simulink model "Assembly_For_Simscape"  (R2023b)
settings: Solver=VariableStepAuto  StartTime=0.0  StopTime=38  RelTol=1e-3
InitFcn:
  | addpath(genpath(pwd));
  | disp('✅ InitFcn executed');
  | Assembly_For_Simscape_DataFile;  % Run the data file script to load smiData
model workspace: external: MAT-File C:\Users\amine\OneDrive - TUM\Desktop\Bachelor Thesis\SIMSCAPE\Simscape files\slprj\sim\varcache\Assembly_For_Simscape\varInfo.mat (data not in the file)
undefined symbols (not defined in the file or in its folder): sigbuilder_block, smiData, X, Y, Z
libraries: sm_lib x76, nesl_utility x32
(part 3 of 3)

== system Assembly_For_Simscape/Project_MiniHex/Stewart_Platform/Horn-BallJoint-Rod-BallJoint 4/ASSEMBLY_Horn_sphere_1_RIGID ==
  ReferenceFrame : sm_lib/Frames and Transforms/Reference Frame
  Solid : sm_lib/Body Elements/File Solid  ExtGeomFileName=ASSEMBLY_Horn_sphere_Default_sldprt.STEP  UnitType=FromFile  ExtGeomFileUnits=m  StepReaderType=HEX  ExportConvexHullGeometry=off  InertiaType=Custom  Mass=smiData.Solid(4).mass  MassUnits=kg  CenterOfMass=smiData.Solid(4).CoM  CenterOfMassUnits=mm  MomentsOfInertia=smiData.Solid(4).MoI  MomentsOfInertiaUnits=kg*mm^2  ProductsOfInertia=smiData.Solid(4).PoI  ProductsOfInertiaUnits=kg*mm^2  BasedOnType=DensityFromFile  Density=1000  DensityUnits=kg/m^3  DoExposeReferenceFrame=off  SerializedFrames=<Frames><Frame><Id>Frame1</Id><Value><Name>horn central frame 2</Name><Origin><Source>GeometricFeature</Source><FeatureName>circular curve 6</FeatureName></Origin><PrimaryAxis><DefinedDirection>+Z</DefinedDirection><Source>CenterOfMassFrame</Source><SourceDirection>-Z</SourceDirection><FeatureName></FeatureName></PrimaryAxis><SecondaryAxis><DefinedDirection>-X</DefinedDirection><Source>CenterOfMassFrame</Source><SourceDirection>+X</SourceDirection><FeatureName></FeatureName></SecondaryAxis></Value></Frame><Frame><Id>Frame2</Id><Value><Name>horn outer frame 2</Name><Origin><Source>GeometricFeature</Source><FeatureName>circular curve 79</FeatureName></Origin><PrimaryAxis><DefinedDirection>+Z</DefinedDirection><Source>CenterOfMassFrame</Source><SourceDirection>-Z</SourceDirection><FeatureName></FeatureName></PrimaryAxis><SecondaryAxis><DefinedDirection>+X</DefinedDirection><Source>GeometricFeature</Source><SourceDirection>+X</SourceDirection><FeatureName>circular curve 79</FeatureName></SecondaryAxis></Value></Frame><Frame><Id>Frame3</Id><Value><Name>COG</Name><Origin><Source>CenterOfMassFrame</Source><FeatureName></FeatureName></Origin><PrimaryAxis><DefinedDirection>-Z</DefinedDirection><Source>GeometricFeature</Source><SourceDirection>+Z</SourceDirection><FeatureName>planar surface 3</FeatureName></PrimaryAxis><SecondaryAxis><DefinedDirection>+X</DefinedDirection><Source>CenterOfMassFrame</Source><SourceDirection>+X</SourceDirection><FeatureName></FeatureName></SecondaryAxis></Value></Frame></Frames>  GraphicType=FromGeometry  MarkerShape=Sphere  MarkerSize=10  GraphicVisPropType=SimpleVisualProperties  GraphicDiffuseColor=smiData.Solid(4).color  GraphicSpecularColor=[0.5 0.5 0.5 1.0]  GraphicAmbientColor=[0.15 0.15 0.15 1.0]  GraphicEmissiveColor=[0.0 0.0 0.0 1.0]  GraphicShininess=75  GraphicOpacity=smiData.Solid(4).opacity
  F2 : PMIOPort  Side=Left
  F1 : PMIOPort  Port=2  Side=Left
  F : PMIOPort  Port=3  Side=Left
  connections:
  ReferenceFrame/RConn1 -- F2/RConn1 -- Solid/LConn2
  Solid/LConn1 -- F1/RConn1
  Solid/RConn1 -- F/RConn1

== system Assembly_For_Simscape/Project_MiniHex/Stewart_Platform/Horn-BallJoint-Rod-BallJoint 4/Ball_Joint_3mm_outer_sphere_2_RIGID ==
  ReferenceFrame : sm_lib/Frames and Transforms/Reference Frame
  Solid : sm_lib/Body Elements/File Solid  ExtGeomFileName=Ball Joint 3mm outer sphere_Default_sldprt.STEP  UnitType=FromFile  ExtGeomFileUnits=m  StepReaderType=HEX  ExportConvexHullGeometry=off  InertiaType=Custom  Mass=smiData.Solid(5).mass  MassUnits=kg  CenterOfMass=smiData.Solid(5).CoM  CenterOfMassUnits=mm  MomentsOfInertia=smiData.Solid(5).MoI  MomentsOfInertiaUnits=kg*mm^2  ProductsOfInertia=smiData.Solid(5).PoI  ProductsOfInertiaUnits=kg*mm^2  BasedOnType=DensityFromFile  Density=1000  DensityUnits=kg/m^3  DoExposeReferenceFrame=on  SerializedFrames=<Frames><Frame><Id>Frame1</Id><Value><Name>ball joint center</Name><Origin><Source>GeometricFeature</Source><FeatureName>spherical surface 4</FeatureName></Origin><PrimaryAxis><DefinedDirection>+Z</DefinedDirection><Source>GeometricFeature</Source><SourceDirection>+Z</SourceDirection><FeatureName>circular curve 27</FeatureName></PrimaryAxis><SecondaryAxis><DefinedDirection>-Y</DefinedDirection><Source>ReferenceFrame</Source><SourceDirection>+Y</SourceDirection><FeatureName></FeatureName></SecondaryAxis></Value></Frame><Frame><Id>Frame2</Id><Value><Name>Rod rotation link</Name><Origin><Source>GeometricFeature</Source><FeatureName>planar surface 3</FeatureName></Origin><PrimaryAxis><DefinedDirection>+Z</DefinedDirection><Source>GeometricFeature</Source><SourceDirection>+Z</SourceDirection><FeatureName>planar surface 3</FeatureName></PrimaryAxis><SecondaryAxis><DefinedDirection>+X</DefinedDirection><Source>ReferenceFrame</Source><SourceDirection>+X</SourceDirection><FeatureName></FeatureName></SecondaryAxis></Value></Frame></Frames>  GraphicType=FromGeometry  MarkerShape=Sphere  MarkerSize=10  GraphicVisPropType=SimpleVisualProperties  GraphicDiffuseColor=smiData.Solid(5).color  GraphicSpecularColor=[0.5 0.5 0.5 1.0]  GraphicAmbientColor=[0.15 0.15 0.15 1.0]  GraphicEmissiveColor=[0.0 0.0 0.0 1.0]  GraphicShininess=75  GraphicOpacity=smiData.Solid(5).opacity
  F : PMIOPort  Side=Left
  F1 : PMIOPort  Port=2  Side=Left
  connections:
  ReferenceFrame/RConn1 -- Solid/RConn1
  Solid/LConn1 -- F/RConn1
  Solid/LConn2 -- F1/RConn1

== system Assembly_For_Simscape/Project_MiniHex/Stewart_Platform/Horn-BallJoint-Rod-BallJoint 4/Ball_Joint_3mm_outer_sphere_2_RIGID2 ==
  ReferenceFrame : sm_lib/Frames and Transforms/Reference Frame
  Solid : sm_lib/Body Elements/File Solid  ExtGeomFileName=Ball Joint 3mm outer sphere_Default_sldprt.STEP  UnitType=FromFile  ExtGeomFileUnits=m  StepReaderType=HEX  ExportConvexHullGeometry=off  InertiaType=Custom  Mass=smiData.Solid(5).mass  MassUnits=kg  CenterOfMass=smiData.Solid(5).CoM  CenterOfMassUnits=mm  MomentsOfInertia=smiData.Solid(5).MoI  MomentsOfInertiaUnits=kg*mm^2  ProductsOfInertia=smiData.Solid(5).PoI  ProductsOfInertiaUnits=kg*mm^2  BasedOnType=DensityFromFile  Density=1000  DensityUnits=kg/m^3  DoExposeReferenceFrame=on  SerializedFrames=<Frames><Frame><Id>Frame1</Id><Value><Name>ball joint center</Name><Origin><Source>GeometricFeature</Source><FeatureName>spherical surface 4</FeatureName></Origin><PrimaryAxis><DefinedDirection>+Z</DefinedDirection><Source>GeometricFeature</Source><SourceDirection>+Z</SourceDirection><FeatureName>circular curve 27</FeatureName></PrimaryAxis><SecondaryAxis><DefinedDirection>-Y</DefinedDirection><Source>ReferenceFrame</Source><SourceDirection>+Y</SourceDirection><FeatureName></FeatureName></SecondaryAxis></Value></Frame><Frame><Id>Frame2</Id><Value><Name>Rod rotation link</Name><Origin><Source>GeometricFeature</Source><FeatureName>planar surface 3</FeatureName></Origin><PrimaryAxis><DefinedDirection>+Z</DefinedDirection><Source>GeometricFeature</Source><SourceDirection>+Z</SourceDirection><FeatureName>planar surface 3</FeatureName></PrimaryAxis><SecondaryAxis><DefinedDirection>+X</DefinedDirection><Source>ReferenceFrame</Source><SourceDirection>+X</SourceDirection><FeatureName></FeatureName></SecondaryAxis></Value></Frame></Frames>  GraphicType=FromGeometry  MarkerShape=Sphere  MarkerSize=10  GraphicVisPropType=SimpleVisualProperties  GraphicDiffuseColor=smiData.Solid(5).color  GraphicSpecularColor=[0.5 0.5 0.5 1.0]  GraphicAmbientColor=[0.15 0.15 0.15 1.0]  GraphicEmissiveColor=[0.0 0.0 0.0 1.0]  GraphicShininess=75  GraphicOpacity=smiData.Solid(5).opacity
  F : PMIOPort  Side=Left
  F1 : PMIOPort  Port=2  Side=Right
  connections:
  ReferenceFrame/RConn1 -- Solid/RConn1
  Solid/LConn1 -- F/RConn1
  Solid/LConn2 -- F1/RConn1

== system Assembly_For_Simscape/Project_MiniHex/Stewart_Platform/Horn-BallJoint-Rod-BallJoint 4/Rod_1_RIGID ==
  ReferenceFrame : sm_lib/Frames and Transforms/Reference Frame
  Solid : sm_lib/Body Elements/File Solid  ExtGeomFileName=Rod_Default_sldprt.STEP  UnitType=FromFile  ExtGeomFileUnits=m  StepReaderType=HEX  ExportConvexHullGeometry=off  InertiaType=Custom  Mass=smiData.Solid(3).mass  MassUnits=kg  CenterOfMass=smiData.Solid(3).CoM  CenterOfMassUnits=m  MomentsOfInertia=smiData.Solid(3).MoI  MomentsOfInertiaUnits=kg*m^2  ProductsOfInertia=smiData.Solid(3).PoI  ProductsOfInertiaUnits=kg*m^2  BasedOnType=DensityFromFile  Density=1000  DensityUnits=kg/m^3  DoExposeReferenceFrame=on  SerializedFrames=<Frames><Frame><Id>Frame1</Id><Value><Name>F1</Name><Origin><Source>GeometricFeature</Source><FeatureName>planar surface 4</FeatureName></Origin><PrimaryAxis><DefinedDirection>-Z</DefinedDirection><Source>GeometricFeature</Source><SourceDirection>+Z</SourceDirection><FeatureName>planar surface 4</FeatureName></PrimaryAxis><SecondaryAxis><DefinedDirection>+X</DefinedDirection><Source>ReferenceFrame</Source><SourceDirection>+X</SourceDirection><FeatureName></FeatureName></SecondaryAxis></Value></Frame><Frame><Id>Frame2</Id><Value><Name>F2</Name><Origin><Source>GeometricFeature</Source><FeatureName>planar surface 3</FeatureName></Origin><PrimaryAxis><DefinedDirection>-Z</DefinedDirection><Source>CenterOfMassFrame</Source><SourceDirection>+Y</SourceDirection><FeatureName></FeatureName></PrimaryAxis><SecondaryAxis><DefinedDirection>+Y</DefinedDirection><Source>CenterOfMassFrame</Source><SourceDirection>+Z</SourceDirection><FeatureName></FeatureName></SecondaryAxis></Value></Frame></Frames>  GraphicType=FromGeometry  MarkerShape=Sphere  MarkerSize=10  GraphicVisPropType=SimpleVisualProperties  GraphicDiffuseColor=smiData.Solid(3).color  GraphicSpecularColor=[0.5 0.5 0.5 1.0]  GraphicAmbientColor=[0.15 0.15 0.15 1.0]  GraphicEmissiveColor=[0.0 0.0 0.0 1.0]  GraphicShininess=75  GraphicOpacity=smiData.Solid(3).opacity
  F : PMIOPort  Side=Left
  F1 : PMIOPort  Port=2  Side=Right
  connections:
  ReferenceFrame/RConn1 -- Solid/RConn1
  Solid/LConn1 -- F/RConn1
  Solid/LConn2 -- F1/RConn1

== system Assembly_For_Simscape/Project_MiniHex/Stewart_Platform/Horn-BallJoint-Rod-BallJoint 5/ASSEMBLY_Horn_sphere_1_RIGID ==
  ReferenceFrame : sm_lib/Frames and Transforms/Reference Frame
  Solid : sm_lib/Body Elements/File Solid  ExtGeomFileName=ASSEMBLY_Horn_sphere_Default_sldprt.STEP  UnitType=FromFile  ExtGeomFileUnits=m  StepReaderType=HEX  ExportConvexHullGeometry=off  InertiaType=Custom  Mass=smiData.Solid(4).mass  MassUnits=kg  CenterOfMass=smiData.Solid(4).CoM  CenterOfMassUnits=mm  MomentsOfInertia=smiData.Solid(4).MoI  MomentsOfInertiaUnits=kg*mm^2  ProductsOfInertia=smiData.Solid(4).PoI  ProductsOfInertiaUnits=kg*mm^2  BasedOnType=DensityFromFile  Density=1000  DensityUnits=kg/m^3  DoExposeReferenceFrame=off  SerializedFrames=<Frames><Frame><Id>Frame1</Id><Value><Name>horn central frame</Name><Origin><Source>GeometricFeature</Source><FeatureName>circular curve 6</FeatureName></Origin><PrimaryAxis><DefinedDirection>+Z</DefinedDirection><Source>CenterOfMassFrame</Source><SourceDirection>-Z</SourceDirection><FeatureName></FeatureName></PrimaryAxis><SecondaryAxis><DefinedDirection>-X</DefinedDirection><Source>CenterOfMassFrame</Source><SourceDirection>-X</SourceDirection><FeatureName></FeatureName></SecondaryAxis></Value></Frame><Frame><Id>Frame2</Id><Value><Name>horn outer frame </Name><Origin><Source>GeometricFeature</Source><FeatureName>circular curve 79</FeatureName></Origin><PrimaryAxis><DefinedDirection>+Z</DefinedDirection><Source>CenterOfMassFrame</Source><SourceDirection>-Z</SourceDirection><FeatureName></FeatureName></PrimaryAxis><SecondaryAxis><DefinedDirection>-X</DefinedDirection><Source>GeometricFeature</Source><SourceDirection>+X</SourceDirection><FeatureName>circular curve 79</FeatureName></SecondaryAxis></Value></Frame><Frame><Id>Frame3</Id><Value><Name>COG</Name><Origin><Source>CenterOfMassFrame</Source><FeatureName></FeatureName></Origin><PrimaryAxis><DefinedDirection>-Z</DefinedDirection><Source>GeometricFeature</Source><SourceDirection>+Z</SourceDirection><FeatureName>planar surface 3</FeatureName></PrimaryAxis><SecondaryAxis><DefinedDirection>+X</DefinedDirection><Source>CenterOfMassFrame</Source><SourceDirection>+X</SourceDirection><FeatureName></FeatureName></SecondaryAxis></Value></Frame></Frames>  GraphicType=FromGeometry  MarkerShape=Sphere  MarkerSize=10  GraphicVisPropType=SimpleVisualProperties  GraphicDiffuseColor=smiData.Solid(4).color  GraphicSpecularColor=[0.5 0.5 0.5 1.0]  GraphicAmbientColor=[0.15 0.15 0.15 1.0]  GraphicEmissiveColor=[0.0 0.0 0.0 1.0]  GraphicShininess=75  GraphicOpacity=smiData.Solid(4).opacity
  F2 : PMIOPort  Side=Left
  F1 : PMIOPort  Port=2  Side=Left
  F : PMIOPort  Port=3  Side=Left
  connections:
  ReferenceFrame/RConn1 -- Solid/LConn2 -- F2/RConn1
  Solid/LConn1 -- F1/RConn1
  Solid/RConn1 -- F/RConn1

== system Assembly_For_Simscape/Project_MiniHex/Stewart_Platform/Horn-BallJoint-Rod-BallJoint 5/Ball_Joint_3mm_outer_sphere_2_RIGID ==
  ReferenceFrame : sm_lib/Frames and Transforms/Reference Frame
  Solid : sm_lib/Body Elements/File Solid  ExtGeomFileName=Ball Joint 3mm outer sphere_Default_sldprt.STEP  UnitType=FromFile  ExtGeomFileUnits=m  StepReaderType=HEX  ExportConvexHullGeometry=off  InertiaType=Custom  Mass=smiData.Solid(5).mass  MassUnits=kg  CenterOfMass=smiData.Solid(5).CoM  CenterOfMassUnits=mm  MomentsOfInertia=smiData.Solid(5).MoI  MomentsOfInertiaUnits=kg*mm^2  ProductsOfInertia=smiData.Solid(5).PoI  ProductsOfInertiaUnits=kg*mm^2  BasedOnType=DensityFromFile  Density=1000  DensityUnits=kg/m^3  DoExposeReferenceFrame=on  SerializedFrames=<Frames><Frame><Id>Frame1</Id><Value><Name>ball joint center</Name><Origin><Source>GeometricFeature</Source><FeatureName>spherical surface 4</FeatureName></Origin><PrimaryAxis><DefinedDirection>+Z</DefinedDirection><Source>GeometricFeature</Source><SourceDirection>+Z</SourceDirection><FeatureName>circular curve 27</FeatureName></PrimaryAxis><SecondaryAxis><DefinedDirection>-Y</DefinedDirection><Source>ReferenceFrame</Source><SourceDirection>+Y</SourceDirection><FeatureName></FeatureName></SecondaryAxis></Value></Frame><Frame><Id>Frame2</Id><Value><Name>Rod rotation link</Name><Origin><Source>GeometricFeature</Source><FeatureName>planar surface 3</FeatureName></Origin><PrimaryAxis><DefinedDirection>+Z</DefinedDirection><Source>GeometricFeature</Source><SourceDirection>+Z</SourceDirection><FeatureName>planar surface 3</FeatureName></PrimaryAxis><SecondaryAxis><DefinedDirection>+X</DefinedDirection><Source>ReferenceFrame</Source><SourceDirection>+X</SourceDirection><FeatureName></FeatureName></SecondaryAxis></Value></Frame></Frames>  GraphicType=FromGeometry  MarkerShape=Sphere  MarkerSize=10  GraphicVisPropType=SimpleVisualProperties  GraphicDiffuseColor=smiData.Solid(5).color  GraphicSpecularColor=[0.5 0.5 0.5 1.0]  GraphicAmbientColor=[0.15 0.15 0.15 1.0]  GraphicEmissiveColor=[0.0 0.0 0.0 1.0]  GraphicShininess=75  GraphicOpacity=smiData.Solid(5).opacity
  F : PMIOPort  Side=Left
  F1 : PMIOPort  Port=2  Side=Left
  connections:
  ReferenceFrame/RConn1 -- Solid/RConn1
  Solid/LConn1 -- F/RConn1
  Solid/LConn2 -- F1/RConn1

== system Assembly_For_Simscape/Project_MiniHex/Stewart_Platform/Horn-BallJoint-Rod-BallJoint 5/Ball_Joint_3mm_outer_sphere_2_RIGID2 ==
  ReferenceFrame : sm_lib/Frames and Transforms/Reference Frame
  Solid : sm_lib/Body Elements/File Solid  ExtGeomFileName=Ball Joint 3mm outer sphere_Default_sldprt.STEP  UnitType=FromFile  ExtGeomFileUnits=m  StepReaderType=HEX  ExportConvexHullGeometry=off  InertiaType=Custom  Mass=smiData.Solid(5).mass  MassUnits=kg  CenterOfMass=smiData.Solid(5).CoM  CenterOfMassUnits=mm  MomentsOfInertia=smiData.Solid(5).MoI  MomentsOfInertiaUnits=kg*mm^2  ProductsOfInertia=smiData.Solid(5).PoI  ProductsOfInertiaUnits=kg*mm^2  BasedOnType=DensityFromFile  Density=1000  DensityUnits=kg/m^3  DoExposeReferenceFrame=on  SerializedFrames=<Frames><Frame><Id>Frame1</Id><Value><Name>ball joint center</Name><Origin><Source>GeometricFeature</Source><FeatureName>spherical surface 4</FeatureName></Origin><PrimaryAxis><DefinedDirection>+Z</DefinedDirection><Source>GeometricFeature</Source><SourceDirection>+Z</SourceDirection><FeatureName>circular curve 27</FeatureName></PrimaryAxis><SecondaryAxis><DefinedDirection>-Y</DefinedDirection><Source>ReferenceFrame</Source><SourceDirection>+Y</SourceDirection><FeatureName></FeatureName></SecondaryAxis></Value></Frame><Frame><Id>Frame2</Id><Value><Name>Rod rotation link</Name><Origin><Source>GeometricFeature</Source><FeatureName>planar surface 3</FeatureName></Origin><PrimaryAxis><DefinedDirection>+Z</DefinedDirection><Source>GeometricFeature</Source><SourceDirection>+Z</SourceDirection><FeatureName>planar surface 3</FeatureName></PrimaryAxis><SecondaryAxis><DefinedDirection>+X</DefinedDirection><Source>ReferenceFrame</Source><SourceDirection>+X</SourceDirection><FeatureName></FeatureName></SecondaryAxis></Value></Frame></Frames>  GraphicType=FromGeometry  MarkerShape=Sphere  MarkerSize=10  GraphicVisPropType=SimpleVisualProperties  GraphicDiffuseColor=smiData.Solid(5).color  GraphicSpecularColor=[0.5 0.5 0.5 1.0]  GraphicAmbientColor=[0.15 0.15 0.15 1.0]  GraphicEmissiveColor=[0.0 0.0 0.0 1.0]  GraphicShininess=75  GraphicOpacity=smiData.Solid(5).opacity
  F : PMIOPort  Side=Left
  F1 : PMIOPort  Port=2  Side=Right
  connections:
  ReferenceFrame/RConn1 -- Solid/RConn1
  Solid/LConn1 -- F/RConn1
  Solid/LConn2 -- F1/RConn1

== system Assembly_For_Simscape/Project_MiniHex/Stewart_Platform/Horn-BallJoint-Rod-BallJoint 5/Rod_1_RIGID ==
  ReferenceFrame : sm_lib/Frames and Transforms/Reference Frame
  Solid : sm_lib/Body Elements/File Solid  ExtGeomFileName=Rod_Default_sldprt.STEP  UnitType=FromFile  ExtGeomFileUnits=m  StepReaderType=HEX  ExportConvexHullGeometry=off  InertiaType=Custom  Mass=smiData.Solid(3).mass  MassUnits=kg  CenterOfMass=smiData.Solid(3).CoM  CenterOfMassUnits=m  MomentsOfInertia=smiData.Solid(3).MoI  MomentsOfInertiaUnits=kg*m^2  ProductsOfInertia=smiData.Solid(3).PoI  ProductsOfInertiaUnits=kg*m^2  BasedOnType=DensityFromFile  Density=1000  DensityUnits=kg/m^3  DoExposeReferenceFrame=on  SerializedFrames=<Frames><Frame><Id>Frame1</Id><Value><Name>F1</Name><Origin><Source>GeometricFeature</Source><FeatureName>planar surface 4</FeatureName></Origin><PrimaryAxis><DefinedDirection>-Z</DefinedDirection><Source>GeometricFeature</Source><SourceDirection>+Z</SourceDirection><FeatureName>planar surface 4</FeatureName></PrimaryAxis><SecondaryAxis><DefinedDirection>+X</DefinedDirection><Source>ReferenceFrame</Source><SourceDirection>+X</SourceDirection><FeatureName></FeatureName></SecondaryAxis></Value></Frame><Frame><Id>Frame2</Id><Value><Name>F2</Name><Origin><Source>GeometricFeature</Source><FeatureName>planar surface 3</FeatureName></Origin><PrimaryAxis><DefinedDirection>-Z</DefinedDirection><Source>CenterOfMassFrame</Source><SourceDirection>+Y</SourceDirection><FeatureName></FeatureName></PrimaryAxis><SecondaryAxis><DefinedDirection>+Y</DefinedDirection><Source>CenterOfMassFrame</Source><SourceDirection>+Z</SourceDirection><FeatureName></FeatureName></SecondaryAxis></Value></Frame></Frames>  GraphicType=FromGeometry  MarkerShape=Sphere  MarkerSize=10  GraphicVisPropType=SimpleVisualProperties  GraphicDiffuseColor=smiData.Solid(3).color  GraphicSpecularColor=[0.5 0.5 0.5 1.0]  GraphicAmbientColor=[0.15 0.15 0.15 1.0]  GraphicEmissiveColor=[0.0 0.0 0.0 1.0]  GraphicShininess=75  GraphicOpacity=smiData.Solid(3).opacity
  F : PMIOPort  Side=Left
  F1 : PMIOPort  Port=2  Side=Right
  connections:
  ReferenceFrame/RConn1 -- Solid/RConn1
  Solid/LConn1 -- F/RConn1
  Solid/LConn2 -- F1/RConn1

== system Assembly_For_Simscape/Project_MiniHex/Stewart_Platform/Horn-BallJoint-Rod-BallJoint 6/ASSEMBLY_Horn_sphere_1_RIGID ==
  ReferenceFrame : sm_lib/Frames and Transforms/Reference Frame
  Solid : sm_lib/Body Elements/File Solid  ExtGeomFileName=ASSEMBLY_Horn_sphere_Default_sldprt.STEP  UnitType=FromFile  ExtGeomFileUnits=m  StepReaderType=HEX  ExportConvexHullGeometry=off  InertiaType=Custom  Mass=smiData.Solid(4).mass  MassUnits=kg  CenterOfMass=smiData.Solid(4).CoM  CenterOfMassUnits=mm  MomentsOfInertia=smiData.Solid(4).MoI  MomentsOfInertiaUnits=kg*mm^2  ProductsOfInertia=smiData.Solid(4).PoI  ProductsOfInertiaUnits=kg*mm^2  BasedOnType=DensityFromFile  Density=1000  DensityUnits=kg/m^3  DoExposeReferenceFrame=off  SerializedFrames=<Frames><Frame><Id>Frame1</Id><Value><Name>horn central frame 2</Name><Origin><Source>GeometricFeature</Source><FeatureName>circular curve 6</FeatureName></Origin><PrimaryAxis><DefinedDirection>+Z</DefinedDirection><Source>CenterOfMassFrame</Source><SourceDirection>-Z</SourceDirection><FeatureName></FeatureName></PrimaryAxis><SecondaryAxis><DefinedDirection>-X</DefinedDirection><Source>CenterOfMassFrame</Source><SourceDirection>+X</SourceDirection><FeatureName></FeatureName></SecondaryAxis></Value></Frame><Frame><Id>Frame2</Id><Value><Name>horn outer frame 2</Name><Origin><Source>GeometricFeature</Source><FeatureName>circular curve 79</FeatureName></Origin><PrimaryAxis><DefinedDirection>+Z</DefinedDirection><Source>CenterOfMassFrame</Source><SourceDirection>-Z</SourceDirection><FeatureName></FeatureName></PrimaryAxis><SecondaryAxis><DefinedDirection>+X</DefinedDirection><Source>GeometricFeature</Source><SourceDirection>+X</SourceDirection><FeatureName>circular curve 79</FeatureName></SecondaryAxis></Value></Frame><Frame><Id>Frame3</Id><Value><Name>COG</Name><Origin><Source>CenterOfMassFrame</Source><FeatureName></FeatureName></Origin><PrimaryAxis><DefinedDirection>-Z</DefinedDirection><Source>GeometricFeature</Source><SourceDirection>+Z</SourceDirection><FeatureName>planar surface 3</FeatureName></PrimaryAxis><SecondaryAxis><DefinedDirection>+X</DefinedDirection><Source>CenterOfMassFrame</Source><SourceDirection>+X</SourceDirection><FeatureName></FeatureName></SecondaryAxis></Value></Frame></Frames>  GraphicType=FromGeometry  MarkerShape=Sphere  MarkerSize=10  GraphicVisPropType=SimpleVisualProperties  GraphicDiffuseColor=smiData.Solid(4).color  GraphicSpecularColor=[0.5 0.5 0.5 1.0]  GraphicAmbientColor=[0.15 0.15 0.15 1.0]  GraphicEmissiveColor=[0.0 0.0 0.0 1.0]  GraphicShininess=75  GraphicOpacity=smiData.Solid(4).opacity
  F2 : PMIOPort  Side=Left
  F1 : PMIOPort  Port=2  Side=Left
  F : PMIOPort  Port=3  Side=Left
  connections:
  ReferenceFrame/RConn1 -- F2/RConn1 -- Solid/LConn2
  Solid/LConn1 -- F1/RConn1
  Solid/RConn1 -- F/RConn1

== system Assembly_For_Simscape/Project_MiniHex/Stewart_Platform/Horn-BallJoint-Rod-BallJoint 6/Ball_Joint_3mm_outer_sphere_2_RIGID ==
  ReferenceFrame : sm_lib/Frames and Transforms/Reference Frame
  Solid : sm_lib/Body Elements/File Solid  ExtGeomFileName=Ball Joint 3mm outer sphere_Default_sldprt.STEP  UnitType=FromFile  ExtGeomFileUnits=m  StepReaderType=HEX  ExportConvexHullGeometry=off  InertiaType=Custom  Mass=smiData.Solid(5).mass  MassUnits=kg  CenterOfMass=smiData.Solid(5).CoM  CenterOfMassUnits=mm  MomentsOfInertia=smiData.Solid(5).MoI  MomentsOfInertiaUnits=kg*mm^2  ProductsOfInertia=smiData.Solid(5).PoI  ProductsOfInertiaUnits=kg*mm^2  BasedOnType=DensityFromFile  Density=1000  DensityUnits=kg/m^3  DoExposeReferenceFrame=on  SerializedFrames=<Frames><Frame><Id>Frame1</Id><Value><Name>ball joint center</Name><Origin><Source>GeometricFeature</Source><FeatureName>spherical surface 4</FeatureName></Origin><PrimaryAxis><DefinedDirection>+Z</DefinedDirection><Source>GeometricFeature</Source><SourceDirection>+Z</SourceDirection><FeatureName>circular curve 27</FeatureName></PrimaryAxis><SecondaryAxis><DefinedDirection>-Y</DefinedDirection><Source>ReferenceFrame</Source><SourceDirection>+Y</SourceDirection><FeatureName></FeatureName></SecondaryAxis></Value></Frame><Frame><Id>Frame2</Id><Value><Name>Rod rotation link</Name><Origin><Source>GeometricFeature</Source><FeatureName>planar surface 3</FeatureName></Origin><PrimaryAxis><DefinedDirection>+Z</DefinedDirection><Source>GeometricFeature</Source><SourceDirection>+Z</SourceDirection><FeatureName>planar surface 3</FeatureName></PrimaryAxis><SecondaryAxis><DefinedDirection>+X</DefinedDirection><Source>ReferenceFrame</Source><SourceDirection>+X</SourceDirection><FeatureName></FeatureName></SecondaryAxis></Value></Frame></Frames>  GraphicType=FromGeometry  MarkerShape=Sphere  MarkerSize=10  GraphicVisPropType=SimpleVisualProperties  GraphicDiffuseColor=smiData.Solid(5).color  GraphicSpecularColor=[0.5 0.5 0.5 1.0]  GraphicAmbientColor=[0.15 0.15 0.15 1.0]  GraphicEmissiveColor=[0.0 0.0 0.0 1.0]  GraphicShininess=75  GraphicOpacity=smiData.Solid(5).opacity
  F : PMIOPort  Side=Left
  F1 : PMIOPort  Port=2  Side=Left
  connections:
  ReferenceFrame/RConn1 -- Solid/RConn1
  Solid/LConn1 -- F/RConn1
  Solid/LConn2 -- F1/RConn1

== system Assembly_For_Simscape/Project_MiniHex/Stewart_Platform/Horn-BallJoint-Rod-BallJoint 6/Ball_Joint_3mm_outer_sphere_2_RIGID2 ==
  ReferenceFrame : sm_lib/Frames and Transforms/Reference Frame
  Solid : sm_lib/Body Elements/File Solid  ExtGeomFileName=Ball Joint 3mm outer sphere_Default_sldprt.STEP  UnitType=FromFile  ExtGeomFileUnits=m  StepReaderType=HEX  ExportConvexHullGeometry=off  InertiaType=Custom  Mass=smiData.Solid(5).mass  MassUnits=kg  CenterOfMass=smiData.Solid(5).CoM  CenterOfMassUnits=mm  MomentsOfInertia=smiData.Solid(5).MoI  MomentsOfInertiaUnits=kg*mm^2  ProductsOfInertia=smiData.Solid(5).PoI  ProductsOfInertiaUnits=kg*mm^2  BasedOnType=DensityFromFile  Density=1000  DensityUnits=kg/m^3  DoExposeReferenceFrame=on  SerializedFrames=<Frames><Frame><Id>Frame1</Id><Value><Name>ball joint center</Name><Origin><Source>GeometricFeature</Source><FeatureName>spherical surface 4</FeatureName></Origin><PrimaryAxis><DefinedDirection>+Z</DefinedDirection><Source>GeometricFeature</Source><SourceDirection>+Z</SourceDirection><FeatureName>circular curve 27</FeatureName></PrimaryAxis><SecondaryAxis><DefinedDirection>-Y</DefinedDirection><Source>ReferenceFrame</Source><SourceDirection>+Y</SourceDirection><FeatureName></FeatureName></SecondaryAxis></Value></Frame><Frame><Id>Frame2</Id><Value><Name>Rod rotation link</Name><Origin><Source>GeometricFeature</Source><FeatureName>planar surface 3</FeatureName></Origin><PrimaryAxis><DefinedDirection>+Z</DefinedDirection><Source>GeometricFeature</Source><SourceDirection>+Z</SourceDirection><FeatureName>planar surface 3</FeatureName></PrimaryAxis><SecondaryAxis><DefinedDirection>+X</DefinedDirection><Source>ReferenceFrame</Source><SourceDirection>+X</SourceDirection><FeatureName></FeatureName></SecondaryAxis></Value></Frame></Frames>  GraphicType=FromGeometry  MarkerShape=Sphere  MarkerSize=10  GraphicVisPropType=SimpleVisualProperties  GraphicDiffuseColor=smiData.Solid(5).color  GraphicSpecularColor=[0.5 0.5 0.5 1.0]  GraphicAmbientColor=[0.15 0.15 0.15 1.0]  GraphicEmissiveColor=[0.0 0.0 0.0 1.0]  GraphicShininess=75  GraphicOpacity=smiData.Solid(5).opacity
  F : PMIOPort  Side=Left
  F1 : PMIOPort  Port=2  Side=Right
  connections:
  ReferenceFrame/RConn1 -- Solid/RConn1
  Solid/LConn1 -- F/RConn1
  Solid/LConn2 -- F1/RConn1

== system Assembly_For_Simscape/Project_MiniHex/Stewart_Platform/Horn-BallJoint-Rod-BallJoint 6/Rod_1_RIGID ==
  ReferenceFrame : sm_lib/Frames and Transforms/Reference Frame
  Solid : sm_lib/Body Elements/File Solid  ExtGeomFileName=Rod_Default_sldprt.STEP  UnitType=FromFile  ExtGeomFileUnits=m  StepReaderType=HEX  ExportConvexHullGeometry=off  InertiaType=Custom  Mass=smiData.Solid(3).mass  MassUnits=kg  CenterOfMass=smiData.Solid(3).CoM  CenterOfMassUnits=m  MomentsOfInertia=smiData.Solid(3).MoI  MomentsOfInertiaUnits=kg*m^2  ProductsOfInertia=smiData.Solid(3).PoI  ProductsOfInertiaUnits=kg*m^2  BasedOnType=DensityFromFile  Density=1000  DensityUnits=kg/m^3  DoExposeReferenceFrame=on  SerializedFrames=<Frames><Frame><Id>Frame1</Id><Value><Name>F1</Name><Origin><Source>GeometricFeature</Source><FeatureName>planar surface 4</FeatureName></Origin><PrimaryAxis><DefinedDirection>-Z</DefinedDirection><Source>GeometricFeature</Source><SourceDirection>+Z</SourceDirection><FeatureName>planar surface 4</FeatureName></PrimaryAxis><SecondaryAxis><DefinedDirection>+X</DefinedDirection><Source>ReferenceFrame</Source><SourceDirection>+X</SourceDirection><FeatureName></FeatureName></SecondaryAxis></Value></Frame><Frame><Id>Frame2</Id><Value><Name>F2</Name><Origin><Source>GeometricFeature</Source><FeatureName>planar surface 3</FeatureName></Origin><PrimaryAxis><DefinedDirection>-Z</DefinedDirection><Source>CenterOfMassFrame</Source><SourceDirection>+Y</SourceDirection><FeatureName></FeatureName></PrimaryAxis><SecondaryAxis><DefinedDirection>+Y</DefinedDirection><Source>CenterOfMassFrame</Source><SourceDirection>+Z</SourceDirection><FeatureName></FeatureName></SecondaryAxis></Value></Frame></Frames>  GraphicType=FromGeometry  MarkerShape=Sphere  MarkerSize=10  GraphicVisPropType=SimpleVisualProperties  GraphicDiffuseColor=smiData.Solid(3).color  GraphicSpecularColor=[0.5 0.5 0.5 1.0]  GraphicAmbientColor=[0.15 0.15 0.15 1.0]  GraphicEmissiveColor=[0.0 0.0 0.0 1.0]  GraphicShininess=75  GraphicOpacity=smiData.Solid(3).opacity
  F : PMIOPort  Side=Left
  F1 : PMIOPort  Port=2  Side=Right
  connections:
  ReferenceFrame/RConn1 -- Solid/RConn1
  Solid/LConn1 -- F/RConn1
  Solid/LConn2 -- F1/RConn1

== matlab function Assembly_For_Simscape/Project_MiniHex/Servo_Angles ==
  data: roll input; servoAngles output; pitch input; yaw input; x input; y input; z input
function servoAngles = stewartBlock(roll, pitch, yaw, x, y, z)
%#codegen

pose = [roll, pitch, yaw, x, y, z];
servoAngles = stewartIK(pose);
servoAngles = reshape(servoAngles, [6, 1]);
end
